simulink model "Robotic_Soldering_Physical"  (R2025b)
settings: Solver=VariableStepAuto  StartTime=0.0  StopTime=10.0  RelTol=1e-3
model workspace (MAT data in the model file):
  Digital = Simulink.ValueType
  Digital.DataType = 'boolean'
  DigitalBus4 = Simulink.Bus
  DigitalBus4.Alignment = -1
  DigitalBus4.PreserveElementDimensions = 0
  DigitalBus4.Elements_internal(1) = Simulink.BusElement
  DigitalBus4.Elements_internal(1).DimensionsMode = 'Fixed'
  DigitalBus4.Elements_internal(1).SamplingMode = 'Sample based'
  DigitalBus4.Elements_internal(1).SampleTime = -1
  DigitalBus4.Elements_internal(1).Name = 'bit1'
  DigitalBus4.Elements_internal(1).DataType_internal = 'double'
  DigitalBus4.Elements_internal(1).Complexity = 'real'
  DigitalBus4.Elements_internal(1).Dimensions = 1
  DigitalBus4.Elements_internal(2) = Simulink.BusElement
  DigitalBus4.Elements_internal(2).DimensionsMode = 'Fixed'
  DigitalBus4.Elements_internal(2).SamplingMode = 'Sample based'
  DigitalBus4.Elements_internal(2).SampleTime = -1
  DigitalBus4.Elements_internal(2).Name = 'bit2'
  DigitalBus4.Elements_internal(2).DataType_internal = 'double'
  DigitalBus4.Elements_internal(2).Complexity = 'real'
  DigitalBus4.Elements_internal(2).Dimensions = 1
  DigitalBus4.Elements_internal(3) = Simulink.BusElement
  DigitalBus4.Elements_internal(3).DimensionsMode = 'Fixed'
  DigitalBus4.Elements_internal(3).SamplingMode = 'Sample based'
  DigitalBus4.Elements_internal(3).SampleTime = -1
  DigitalBus4.Elements_internal(3).Name = 'bit3'
  DigitalBus4.Elements_internal(3).DataType_internal = 'double'
  DigitalBus4.Elements_internal(3).Complexity = 'real'
  DigitalBus4.Elements_internal(3).Dimensions = 1
  DigitalBus4.Elements_internal(4) = Simulink.BusElement
  DigitalBus4.Elements_internal(4).DimensionsMode = 'Fixed'
  DigitalBus4.Elements_internal(4).SamplingMode = 'Sample based'
  DigitalBus4.Elements_internal(4).SampleTime = -1
  DigitalBus4.Elements_internal(4).Name = 'bit4'
  DigitalBus4.Elements_internal(4).DataType_internal = 'double'
  DigitalBus4.Elements_internal(4).Complexity = 'real'
  DigitalBus4.Elements_internal(4).Dimensions = 1
  DigitalBus4.DataScope = 'Auto'
  PWM = Simulink.ValueType
  StepDir = Simulink.ValueType
  VideoStream = Simulink.ValueType
settings Model: Creator=prati  LastModifiedBy=prati

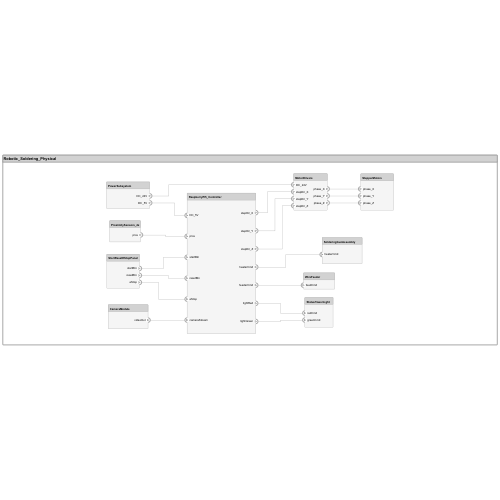
[thumbnail: Simulink's stored preview of the top-level diagram]
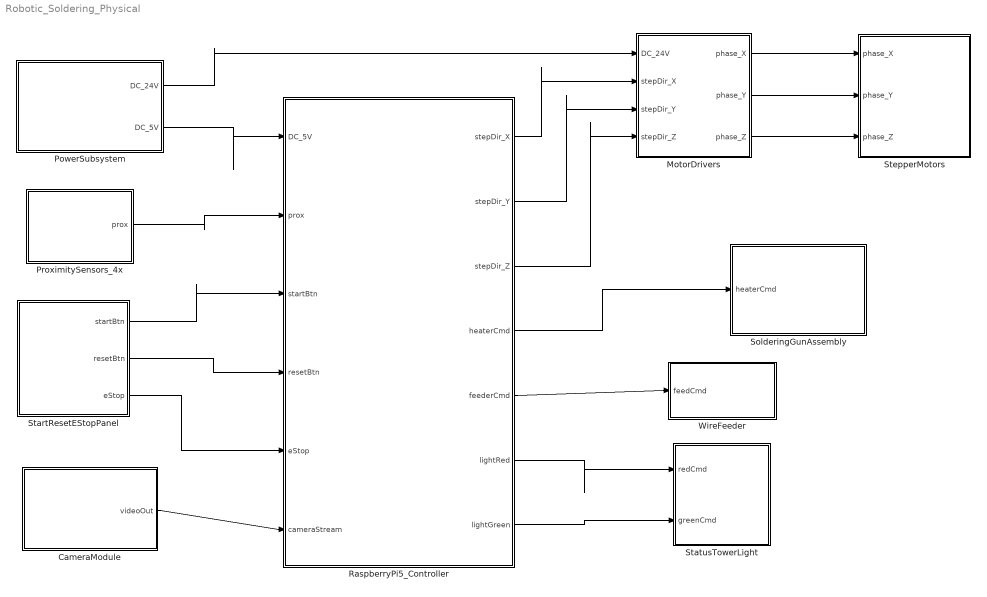
== system Robotic_Soldering_Physical ==
  CameraModule : Subsystem
      settings: PortSchema="{\"entries\":[{\"content\":{\"headerSize\":26,\"margin\":15,\"minimumSpacing\":25,\"sides\":[{\"content\":{},\"type\":\"ConnectorPlacement.EquallySpacedRectSide\",\"uuid\":\"df0712bd-9cd1-4284-b8cc-a563d7d23947\"},{\"content\":{\"connectorIds\":[\"Out1\"],\"side\":\"RIGHT\"},\"type\":\"ConnectorPlacement.EquallySpacedRectSide\",\"uuid\":\"fb1bfffe-10f7-47b0-88bd-447845e3a762\"},{\"content\":{\"side\":\"TOP\"},\"type\":\"ConnectorPlacement.EquallySpacedRectSide\",\"uuid\":\"d4009752-9679-4b5d-9d94-c5d24d63ca5e\"}]},\"type\":\"ConnectorPlacement.EquallySpacedConnector\",\"uuid\":\"7a897207-bb21-4bca-96b0-9aebb9601b63\"}],\"packageUris\":[\"http://schema.mathworks.com/mf0/Connector/R2020b\"],\"version\":\"1.0\"}"
  MotorDrivers : Subsystem
      settings: PortSchema="{\"entries\":[{\"content\":{\"headerSize\":26,\"margin\":15,\"minimumSpacing\":25,\"sides\":[{\"content\":{\"connectorIds\":[\"In1\",\"In2\",\"In3\",\"In4\"]},\"type\":\"ConnectorPlacement.EquallySpacedRectSide\",\"uuid\":\"df0712bd-9cd1-4284-b8cc-a563d7d23947\"},{\"content\":{\"connectorIds\":[\"Out1\",\"Out2\",\"Out3\"],\"side\":\"RIGHT\"},\"type\":\"ConnectorPlacement.EquallySpacedRectSide\",\"uuid\":\"fb1bfffe-10f7-47b0-88bd-447845e3a762\"},{\"content\":{\"side\":\"TOP\"},\"type\":\"ConnectorPlacement.EquallySpacedRectSide\",\"uuid\":\"d4009752-9679-4b5d-9d94-c5d24d63ca5e\"}]},\"type\":\"ConnectorPlacement.EquallySpacedConnector\",\"uuid\":\"7a897207-bb21-4bca-96b0-9aebb9601b63\"}],\"packageUris\":[\"http://schema.mathworks.com/mf0/Connector/R2020b\"],\"version\":\"1.0\"}"
  PowerSubsystem : Subsystem
      settings: PortSchema="{\"entries\":[{\"content\":{\"headerSize\":26,\"margin\":15,\"minimumSpacing\":25,\"sides\":[{\"content\":{},\"type\":\"ConnectorPlacement.EquallySpacedRectSide\",\"uuid\":\"df0712bd-9cd1-4284-b8cc-a563d7d23947\"},{\"content\":{\"connectorIds\":[\"Out1\",\"Out2\"],\"side\":\"RIGHT\"},\"type\":\"ConnectorPlacement.EquallySpacedRectSide\",\"uuid\":\"fb1bfffe-10f7-47b0-88bd-447845e3a762\"},{\"content\":{\"side\":\"TOP\"},\"type\":\"ConnectorPlacement.EquallySpacedRectSide\",\"uuid\":\"d4009752-9679-4b5d-9d94-c5d24d63ca5e\"}]},\"type\":\"ConnectorPlacement.EquallySpacedConnector\",\"uuid\":\"7a897207-bb21-4bca-96b0-9aebb9601b63\"}],\"packageUris\":[\"http://schema.mathworks.com/mf0/Connector/R2020b\"],\"version\":\"1.0\"}"
  ProximitySensors_4x : Subsystem
      settings: PortSchema="{\"entries\":[{\"content\":{\"headerSize\":26,\"margin\":15,\"minimumSpacing\":25,\"sides\":[{\"content\":{},\"type\":\"ConnectorPlacement.EquallySpacedRectSide\",\"uuid\":\"df0712bd-9cd1-4284-b8cc-a563d7d23947\"},{\"content\":{\"connectorIds\":[\"Out1\"],\"side\":\"RIGHT\"},\"type\":\"ConnectorPlacement.EquallySpacedRectSide\",\"uuid\":\"fb1bfffe-10f7-47b0-88bd-447845e3a762\"},{\"content\":{\"side\":\"TOP\"},\"type\":\"ConnectorPlacement.EquallySpacedRectSide\",\"uuid\":\"d4009752-9679-4b5d-9d94-c5d24d63ca5e\"}]},\"type\":\"ConnectorPlacement.EquallySpacedConnector\",\"uuid\":\"7a897207-bb21-4bca-96b0-9aebb9601b63\"}],\"packageUris\":[\"http://schema.mathworks.com/mf0/Connector/R2020b\"],\"version\":\"1.0\"}"
  RaspberryPi5_Controller : Subsystem
      settings: PortSchema="{\"entries\":[{\"content\":{\"headerSize\":26,\"margin\":15,\"minimumSpacing\":25,\"sides\":[{\"content\":{\"connectorIds\":[\"In1\",\"In2\",\"In3\",\"In4\",\"In5\",\"In6\"]},\"type\":\"ConnectorPlacement.EquallySpacedRectSide\",\"uuid\":\"df0712bd-9cd1-4284-b8cc-a563d7d23947\"},{\"content\":{\"connectorIds\":[\"Out1\",\"Out2\",\"Out3\",\"Out4\",\"Out5\",\"Out6\",\"Out7\"],\"side\":\"RIGHT\"},\"type\":\"ConnectorPlacement.EquallySpacedRectSide\",\"uuid\":\"fb1bfffe-10f7-47b0-88bd-447845e3a762\"},{\"content\":{\"side\":\"TOP\"},\"type\":\"ConnectorPlacement.EquallySpacedRectSide\",\"uuid\":\"d4009752-9679-4b5d-9d94-c5d24d63ca5e\"}]},\"type\":\"ConnectorPlacement.EquallySpacedConnector\",\"uuid\":\"7a897207-bb21-4bca-96b0-9aebb9601b63\"}],\"packageUris\":[\"http://schema.mathworks.com/mf0/Connector/R2020b\"],\"version\":\"1.0\"}"
  SolderingGunAssembly : Subsystem
      settings: PortSchema="{\"entries\":[{\"content\":{\"headerSize\":26,\"margin\":15,\"minimumSpacing\":25,\"sides\":[{\"content\":{\"connectorIds\":[\"In1\"]},\"type\":\"ConnectorPlacement.EquallySpacedRectSide\",\"uuid\":\"df0712bd-9cd1-4284-b8cc-a563d7d23947\"},{\"content\":{\"side\":\"RIGHT\"},\"type\":\"ConnectorPlacement.EquallySpacedRectSide\",\"uuid\":\"fb1bfffe-10f7-47b0-88bd-447845e3a762\"},{\"content\":{\"side\":\"TOP\"},\"type\":\"ConnectorPlacement.EquallySpacedRectSide\",\"uuid\":\"d4009752-9679-4b5d-9d94-c5d24d63ca5e\"}]},\"type\":\"ConnectorPlacement.EquallySpacedConnector\",\"uuid\":\"7a897207-bb21-4bca-96b0-9aebb9601b63\"}],\"packageUris\":[\"http://schema.mathworks.com/mf0/Connector/R2020b\"],\"version\":\"1.0\"}"
  StartResetEStopPanel : Subsystem
      settings: PortSchema="{\"entries\":[{\"content\":{\"headerSize\":26,\"margin\":15,\"minimumSpacing\":25,\"sides\":[{\"content\":{},\"type\":\"ConnectorPlacement.EquallySpacedRectSide\",\"uuid\":\"df0712bd-9cd1-4284-b8cc-a563d7d23947\"},{\"content\":{\"connectorIds\":[\"Out1\",\"Out2\",\"Out3\"],\"side\":\"RIGHT\"},\"type\":\"ConnectorPlacement.EquallySpacedRectSide\",\"uuid\":\"fb1bfffe-10f7-47b0-88bd-447845e3a762\"},{\"content\":{\"side\":\"TOP\"},\"type\":\"ConnectorPlacement.EquallySpacedRectSide\",\"uuid\":\"d4009752-9679-4b5d-9d94-c5d24d63ca5e\"}]},\"type\":\"ConnectorPlacement.EquallySpacedConnector\",\"uuid\":\"7a897207-bb21-4bca-96b0-9aebb9601b63\"}],\"packageUris\":[\"http://schema.mathworks.com/mf0/Connector/R2020b\"],\"version\":\"1.0\"}"
  StatusTowerLight : Subsystem
      settings: PortSchema="{\"entries\":[{\"content\":{\"headerSize\":26,\"margin\":15,\"minimumSpacing\":25,\"sides\":[{\"content\":{\"connectorIds\":[\"In1\",\"In2\"]},\"type\":\"ConnectorPlacement.EquallySpacedRectSide\",\"uuid\":\"df0712bd-9cd1-4284-b8cc-a563d7d23947\"},{\"content\":{\"side\":\"RIGHT\"},\"type\":\"ConnectorPlacement.EquallySpacedRectSide\",\"uuid\":\"fb1bfffe-10f7-47b0-88bd-447845e3a762\"},{\"content\":{\"side\":\"TOP\"},\"type\":\"ConnectorPlacement.EquallySpacedRectSide\",\"uuid\":\"d4009752-9679-4b5d-9d94-c5d24d63ca5e\"}]},\"type\":\"ConnectorPlacement.EquallySpacedConnector\",\"uuid\":\"7a897207-bb21-4bca-96b0-9aebb9601b63\"}],\"packageUris\":[\"http://schema.mathworks.com/mf0/Connector/R2020b\"],\"version\":\"1.0\"}"
  StepperMotors : Subsystem
      settings: PortSchema="{\"entries\":[{\"content\":{\"headerSize\":26,\"margin\":15,\"minimumSpacing\":25,\"sides\":[{\"content\":{\"connectorIds\":[\"In1\",\"In2\",\"In3\"]},\"type\":\"ConnectorPlacement.EquallySpacedRectSide\",\"uuid\":\"df0712bd-9cd1-4284-b8cc-a563d7d23947\"},{\"content\":{\"side\":\"RIGHT\"},\"type\":\"ConnectorPlacement.EquallySpacedRectSide\",\"uuid\":\"fb1bfffe-10f7-47b0-88bd-447845e3a762\"},{\"content\":{\"side\":\"TOP\"},\"type\":\"ConnectorPlacement.EquallySpacedRectSide\",\"uuid\":\"d4009752-9679-4b5d-9d94-c5d24d63ca5e\"}]},\"type\":\"ConnectorPlacement.EquallySpacedConnector\",\"uuid\":\"7a897207-bb21-4bca-96b0-9aebb9601b63\"}],\"packageUris\":[\"http://schema.mathworks.com/mf0/Connector/R2020b\"],\"version\":\"1.0\"}"
  WireFeeder : Subsystem
      settings: PortSchema="{\"entries\":[{\"content\":{\"headerSize\":26,\"margin\":15,\"minimumSpacing\":25,\"sides\":[{\"content\":{\"connectorIds\":[\"In1\"]},\"type\":\"ConnectorPlacement.EquallySpacedRectSide\",\"uuid\":\"df0712bd-9cd1-4284-b8cc-a563d7d23947\"},{\"content\":{\"side\":\"RIGHT\"},\"type\":\"ConnectorPlacement.EquallySpacedRectSide\",\"uuid\":\"fb1bfffe-10f7-47b0-88bd-447845e3a762\"},{\"content\":{\"side\":\"TOP\"},\"type\":\"ConnectorPlacement.EquallySpacedRectSide\",\"uuid\":\"d4009752-9679-4b5d-9d94-c5d24d63ca5e\"}]},\"type\":\"ConnectorPlacement.EquallySpacedConnector\",\"uuid\":\"7a897207-bb21-4bca-96b0-9aebb9601b63\"}],\"packageUris\":[\"http://schema.mathworks.com/mf0/Connector/R2020b\"],\"version\":\"1.0\"}"
  wires:
  ProximitySensors_4x/1(prox) -> RaspberryPi5_Controller/2(prox)
  StartResetEStopPanel/3(eStop) -> RaspberryPi5_Controller/5(eStop)
  StartResetEStopPanel/2(resetBtn) -> RaspberryPi5_Controller/4(resetBtn)
  StartResetEStopPanel/1(startBtn) -> RaspberryPi5_Controller/3(startBtn)
  RaspberryPi5_Controller/1(stepDir_X) -> MotorDrivers/2(stepDir_X)
  RaspberryPi5_Controller/2(stepDir_Y) -> MotorDrivers/3(stepDir_Y)
  RaspberryPi5_Controller/3(stepDir_Z) -> MotorDrivers/4(stepDir_Z)
  MotorDrivers/1(phase_X) -> StepperMotors/1(phase_X)
  MotorDrivers/2(phase_Y) -> StepperMotors/2(phase_Y)
  MotorDrivers/3(phase_Z) -> StepperMotors/3(phase_Z)
  RaspberryPi5_Controller/4(heaterCmd) -> SolderingGunAssembly/1(heaterCmd)
  RaspberryPi5_Controller/5(feederCmd) -> WireFeeder/1(feedCmd)
  RaspberryPi5_Controller/6(lightRed) -> StatusTowerLight/1(redCmd)
  RaspberryPi5_Controller/7(lightGreen) -> StatusTowerLight/2(greenCmd)
  CameraModule/1(videoOut) -> RaspberryPi5_Controller/6(cameraStream)
  PowerSubsystem/2(DC_5V) -> RaspberryPi5_Controller/1(DC_5V)
  PowerSubsystem/1(DC_24V) -> MotorDrivers/1(DC_24V)

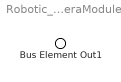
== system Robotic_Soldering_Physical/CameraModule ==
  Bus Element Out1 : Outport  PortName=videoOut

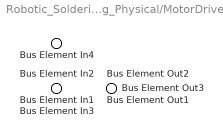
== system Robotic_Soldering_Physical/MotorDrivers ==
  Bus Element In4 : Inport  PortName=DC_24V
  Bus Element In1 : Inport  Port=2  PortName=stepDir_X
  Bus Element In2 : Inport  Port=3  PortName=stepDir_Y
  Bus Element In3 : Inport  Port=4  PortName=stepDir_Z
  Bus Element Out1 : Outport  PortName=phase_X
  Bus Element Out2 : Outport  Port=2  PortName=phase_Y
  Bus Element Out3 : Outport  Port=3  PortName=phase_Z

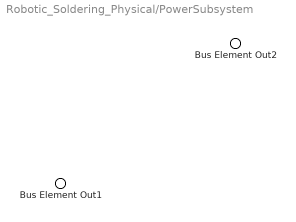
== system Robotic_Soldering_Physical/PowerSubsystem ==
  Bus Element Out2 : Outport  PortName=DC_24V
  Bus Element Out1 : Outport  Port=2  PortName=DC_5V

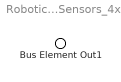
== system Robotic_Soldering_Physical/ProximitySensors_4x ==
  Bus Element Out1 : Outport  PortName=prox

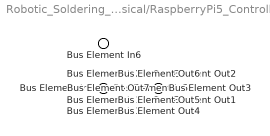
== system Robotic_Soldering_Physical/RaspberryPi5_Controller ==
  Bus Element In6 : Inport  PortName=DC_5V
  Bus Element In1 : Inport  Port=2  PortName=prox
  Bus Element In2 : Inport  Port=3  PortName=startBtn
  Bus Element In3 : Inport  Port=4  PortName=resetBtn
  Bus Element In4 : Inport  Port=5  PortName=eStop
  Bus Element In5 : Inport  Port=6  PortName=cameraStream
  Bus Element Out1 : Outport  PortName=stepDir_X
  Bus Element Out2 : Outport  Port=2  PortName=stepDir_Y
  Bus Element Out3 : Outport  Port=3  PortName=stepDir_Z
  Bus Element Out4 : Outport  Port=4  PortName=heaterCmd
  Bus Element Out5 : Outport  Port=5  PortName=feederCmd
  Bus Element Out6 : Outport  Port=6  PortName=lightRed
  Bus Element Out7 : Outport  Port=7  PortName=lightGreen

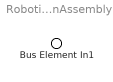
== system Robotic_Soldering_Physical/SolderingGunAssembly ==
  Bus Element In1 : Inport  PortName=heaterCmd

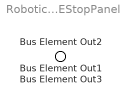
== system Robotic_Soldering_Physical/StartResetEStopPanel ==
  Bus Element Out1 : Outport  PortName=startBtn
  Bus Element Out2 : Outport  Port=2  PortName=resetBtn
  Bus Element Out3 : Outport  Port=3  PortName=eStop

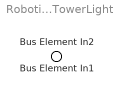
== system Robotic_Soldering_Physical/StatusTowerLight ==
  Bus Element In1 : Inport  PortName=redCmd
  Bus Element In2 : Inport  Port=2  PortName=greenCmd

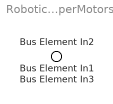
== system Robotic_Soldering_Physical/StepperMotors ==
  Bus Element In1 : Inport  PortName=phase_X
  Bus Element In2 : Inport  Port=2  PortName=phase_Y
  Bus Element In3 : Inport  Port=3  PortName=phase_Z

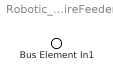
== system Robotic_Soldering_Physical/WireFeeder ==
  Bus Element In1 : Inport  PortName=feedCmd
